simulink model "Drone_swarm_control"  (R2025a)
settings: Solver=FixedStepAuto  StartTime=0.0  StopTime=180  FixedStep=0.001  RelTol=1e-3
InitFcn:
  | %% Simulation parameters and waypoint trajectory
  | % Initial drone positions.
  | init_0=[0;0;0];
  | d_s=4;
  | init_1=init_0+d_s*[-1.1;0.1;0];
  | init_2=init_0+d_s*[0.3;-1.5;0];
  | init_3=init_0+d_s*[1.6;0.4;0];
  | init_4=init_0+d_s*[0.2;1.8;0];
  | 
  | % Initial battery energy in Wh.
  | E_0=77;
  | gain_2=1;
  | 
  | % PID controller gains.
  | PID_p=20;
  | PID_i=50;
  | PID_d=0;
  | 
  | % Router queues and background traffic.
  | router_buffer=160;
  | router_bandwith=300;
  | router_init_queue=[20,0,0,0,0];
  | traffic_mean=20;
  | traffic_variance=1;
  | 
  | % Communication-rate parameters.
  | F_max=2;
  | F_min=0.5;
  | F_H=(F_max+F_min)/3;
  | P_nc=(1-(F_H-F_min)/F_max);
  | 
  | 
  | % Desired formation offsets.
  | init_f_0=[0;0;0];
  | d_f=10;
  | init_f_1=init_0+d_f*[-1;0;0];
  | init_f_2=init_0+d_f*[0;-1;0];
  | init_f_3=init_0+d_f*[1;0;0];
  | init_f_4=init_0+d_f*[0;1;0];
  | 
  | 
  | % Waypoint mission with a fixed cruise altitude.
  | quota_fissa = -20;
  | 
  | waypoints = [
  |       0   0   0   0;
  |      75   0   quota_fissa   0;
  |     150   0   quota_fissa   0;
  |     225   0   quota_fissa   0;
  |     300   0   quota_fissa   0;
  |     300   0   quota_fissa   0;
  |     225  75   quota_fissa   0;
  |     150 150   quota_fissa   0;
  |      75 225   quota_fissa   0;
  |       0 300   quota_fissa   0;
  |       0 300   quota_fissa   0;
  |      75 300   quota_fissa   0;
  |     150 300   quota_fissa   0;
  |     225 300   quota_fissa   0;
  |     300 300   quota_fissa   0;
  |     300 300   quota_fissa   0;
  |     225 225   quota_fissa   0;
  |     150 150   quota_fissa   0;
  |      75  75   quota_fissa   0;
  |       0   0   quota_fissa   0;
  | ];
  | 
  | M = size(waypoints,1);
  | assert(M==20, &apos;You must supply exactly 20 waypoints.&apos;);
  | 
  | % Quadrotor mass and inertia.
  | mass = 1.2;
  | Ib   = diag([1.2416, 1.2416, 2*1.2416]);
  | 
  | % Mission duration and sampling interval.
  | ttot      = 3*60;
  | tdead     = 0;
  | totalTime = ttot + tdead;
  | % Time grid and waypoint trajectory.
  | Ts        = 0.001;
  | Nsamples  = round(totalTime/Ts) + 1;
  | t_sample  = linspace(0, totalTime, Nsamples);
  | 
  | % Waypoint dwell intervals used by the trajectory planner.
  | dwell    = 5;
  | Tflight  = ttot - M*dwell;
  | t_seg    = Tflight/(M-1);
  | 
  | % Repeat waypoint samples at arrival and departure times.
  | t_ext  = zeros(2*M,1);
  | wp_ext = zeros(2*M,4);
  | for i = 1:M
  |     t0             = (i-1)*(t_seg + dwell);
  |     t_ext(2*i-1)   = t0;
  |     t_ext(2*i)     = t0 + dwell;
  |     wp_ext(2*i-1,:)= waypoints(i,:);
  |     wp_ext(2*i,  :)= waypoints(i,:);
  | end
  | 
  | p_d      = zeros(4, Nsamples);
  | dot_p_d  = zeros(4, Nsamples);
  | ddot_p_d = zeros(4, Nsamples);
  | 
  | idx_traj = t_sample <= ttot;
  | t_active = t_sample(idx_traj);
  | 
  | % Build position and yaw splines with zero endpoint velocities.
  | for dim = 1:4
  |     pp   = spline(t_ext, [0, wp_ext(:,dim)&apos;, 0]);
  |     pp1  = fnder(pp,1);
  |     pp2  = fnder(pp,2);
  | 
  |     p_d(dim,    idx_traj) = ppval(pp,  t_active);
  |     dot_p_d(dim,idx_traj) = ppval(pp1, t_active);
  |     ddot_p_d(dim,idx_traj)= ppval(pp2, t_active);
  | end
  | 
  | % Hold the final waypoint during the optional settling interval.
  | if tdead>0
  |     last_wp = waypoints(end,:)&apos;;
  |     p_d(   :, ~idx_traj) = repmat(last_wp, 1, sum(~idx_traj));
  |     dot_p_d(:, ~idx_traj) = 0;
  |     ddot_p_d(:,~idx_traj) = 0;
  | end
  | 
  | % Reference signals used by the Simulink blocks.
  | csi_d      = p_d(1:3, :);
  | psi_d      = p_d(4,   :);
  | dot_csi_d  = dot_p_d(1:3, :);
  | ddot_csi_d = ddot_p_d(1:3, :);
  | dot_psi_d  = dot_p_d(4,   :);
  | ddot_psi_d = ddot_p_d(4,   :);
  | 
  | pos_0     = waypoints(1,1:3);
  | lin_vel_0 = [0 0 0];
  | w_bb_0    = [0 0 0];
  | 
  | 
  | t=t_sample;
undefined symbols (not defined in the file): A_diacenza, DiscIntNeverNeededParam, L
libraries: dspsigops x10, robotcorelib x5, slpidlib x5, dspstat3 x5, simulink x1, uavutilslib x1
(part 1 of 4)
settings Model: Creator=fabioruggiero  LastModifiedBy=tehen
settings ModelReferenceCC: EnableRefExpFcnMdlSchedulingChecks=on
settings RTWCC: GPUComputeCapability=3.5

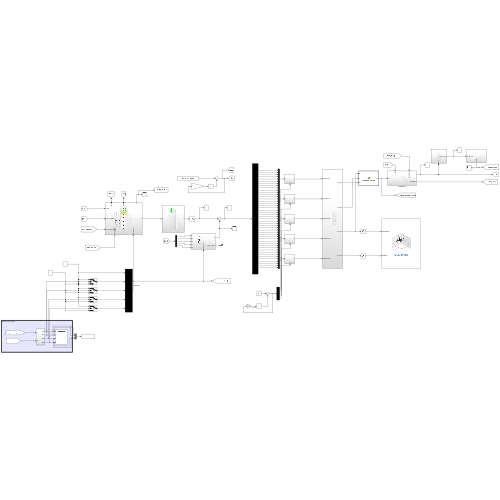
[thumbnail: Simulink's stored preview of the top-level diagram]
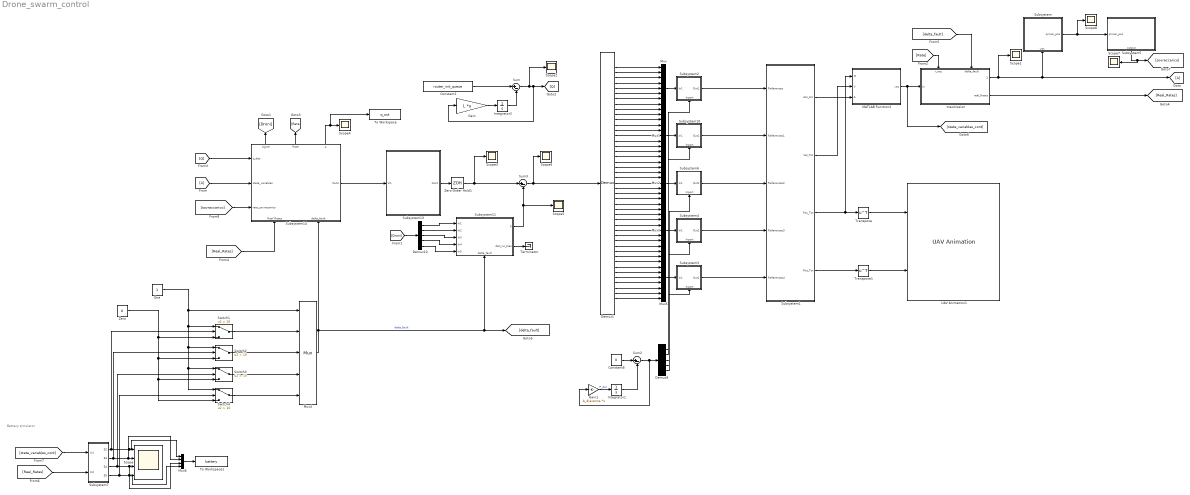
== system Drone_swarm_control ==
  note: Battery simulator
  Constant1 : Constant  Value=router_init_queue
  Constant8 : Constant  Value=0
  Demux1 : Demux  Outputs=45
  Demux10 : Demux  Outputs=5
  Demux9 : Demux  Outputs=5
  From : From
  Gain : Gain  Gain=L  Multiplication=Matrix(K*u)
  Gain1 : Gain  Gain=A_diacenza  Multiplication=Matrix(K*u)
  Goto : Goto
  Integrator1 : Integrator
  Integrator2 : Integrator
  MATLAB Function2 : MATLAB Function  TreatAsAtomicUnit=on
  Mux{,1..3,5} (5 alike) : Mux  Inputs=9
  Mux4 : Mux  Inputs=5
  Mux6 : Mux
  One : Constant  OutDataTypeStr=Inherit: Inherit via back propagation
  Scope : Scope  NumInputPorts=4
      settings: ActiveDisplayYMinimum=73.268572963914167  ActiveDisplayYMaximum=77.414603004009535  DataLoggingVariableName=ScopeData36
  Scope{1..8} (8 alike) : Scope
      Scope1 settings: ActiveDisplayYMinimum=-2.8153611493220492  ActiveDisplayYMaximum=3.6120762005014342  DataLoggingVariableName=ScopeData33
      Scope2 settings: ActiveDisplayYMinimum=-0.80480947223759247  ActiveDisplayYMaximum=7.2432852501383342  DataLoggingVariableName=ScopeData34
      Scope3 settings: ActiveDisplayYMinimum=-143.81794768951772  ActiveDisplayYMaximum=72.930943180534939  DataLoggingVariableName=ScopeData22
      Scope4 settings: ActiveDisplayYMinimum=-19.999999999999996  ActiveDisplayYMaximum=180  DataLoggingVariableName=ScopeData10
      Scope5 settings: ActiveDisplayYMinimum=-31.295142586026412  ActiveDisplayYMaximum=31.13864534366818  DataLoggingVariableName=ScopeData26
      Scope6 settings: ActiveDisplayYMinimum=-63.285546446382227  ActiveDisplayYMaximum=68.103390325053155  DataLoggingVariableName=ScopeData30
      Scope7 settings: ActiveDisplayYMinimum=-1  ActiveDisplayYMaximum=1  DataLoggingVariableName=ScopeData45
      Scope8 settings: ActiveDisplayYMinimum=-34.410281468941783  ActiveDisplayYMaximum=109.69253321204845  DataLoggingVariableName=ScopeData38
  Subsystem : Subsystem
      settings: PortSchema="{\"entries\":[{\"content\":{\"sides\":[{\"content\":{},\"type\":\"ConnectorPlacement.EquallySpacedRectSide\",\"uuid\":\"08878166-f0fb-4fb4-8499-3220f0500d52\"},{\"content\":{\"connectorIds\":[\"Out1\"],\"side\":\"RIGHT\"},\"type\":\"ConnectorPlacement.EquallySpacedRectSide\",\"uuid\":\"3c5bd1ef-4402-434f-96a9-2e68d96c1f89\"},{\"content\":{\"side\":\"TOP\"},\"type\":\"ConnectorPlacement.EquallySpacedRectSide\",\"uuid\":\"fffe2cbe-d1b2-4ad1-ad76-24284be8719f\"},{\"content\":{\"connectorIds\":[\"In1\"],\"side\":\"BOTTOM\"},\"type\":\"ConnectorPlacement.EquallySpacedRectSide\",\"uuid\":\"822b8eda-48e8-4a99-8864-f0043c7d4993\"}]},\"type\":\"ConnectorPlacement.EquallySpacedConnector\",\"uuid\":\"fdf8a493-4def-4212-9b4e-e4f95273dccb\"}],\"packageUris\":[\"http://schema.mathworks.com/mf0/Connector/R2020b\"],\"version\":\"1.0\"}"
  Subsystem1 : Subsystem
  Subsystem10 : Subsystem
      settings: PortSchema="{\"entries\":[{\"content\":{\"sides\":[{\"content\":{\"connectorIds\":[\"In1\"]},\"type\":\"ConnectorPlacement.EquallySpacedRectSide\",\"uuid\":\"6e5d8b99-8054-458f-abbe-7e3d6126420c\"},{\"content\":{\"connectorIds\":[\"Out1\"],\"side\":\"RIGHT\"},\"type\":\"ConnectorPlacement.EquallySpacedRectSide\",\"uuid\":\"d8af8c34-1227-4a19-bfdc-b42d943ed13c\"},{\"content\":{\"side\":\"TOP\"},\"type\":\"ConnectorPlacement.EquallySpacedRectSide\",\"uuid\":\"9c10b933-2873-4349-b535-f2af5c16ec70\"},{\"content\":{\"connectorIds\":[\"In2\"],\"side\":\"BOTTOM\"},\"type\":\"ConnectorPlacement.EquallySpacedRectSide\",\"uuid\":\"05be8d01-ed26-4f96-bcb1-0e501cb43bcc\"}]},\"type\":\"ConnectorPlacement.EquallySpacedConnector\",\"uuid\":\"f87e25de-488b-44c6-b2e5-9d22d609821c\"}],\"packageUris\":[\"http://schema.mathworks.com/mf0/Connector/R2020b\"],\"version\":\"1.0\"}"
  Subsystem11 : Subsystem
      settings: PortSchema="{\"entries\":[{\"content\":{\"sides\":[{\"content\":{\"connectorIds\":[\"In1\",\"In2\",\"In3\",\"In4\",\"In5\"]},\"type\":\"ConnectorPlacement.EquallySpacedRectSide\",\"uuid\":\"82243081-7292-4dd7-bbb8-2b3f3ffda34e\"},{\"content\":{\"connectorIds\":[\"Out1\",\"Out2\"],\"side\":\"RIGHT\"},\"type\":\"ConnectorPlacement.EquallySpacedRectSide\",\"uuid\":\"0c768998-383c-4b1c-86c0-02766a2c634a\"},{\"content\":{\"side\":\"TOP\"},\"type\":\"ConnectorPlacement.EquallySpacedRectSide\",\"uuid\":\"2d16c04a-7161-4b14-a0bc-a057e1fb9d07\"},{\"content\":{\"connectorIds\":[\"In6\"],\"side\":\"BOTTOM\"},\"type\":\"ConnectorPlacement.EquallySpacedRectSide\",\"uuid\":\"700b63a7-d9a8-4585-a364-11c2f92fed84\"}]},\"type\":\"ConnectorPlacement.EquallySpacedConnector\",\"uuid\":\"2c45eea6-509d-46c9-bd27-2690d9a9f219\"}],\"packageUris\":[\"http://schema.mathworks.com/mf0/Connector/R2020b\"],\"version\":\"1.0\"}"
  Subsystem13 : Subsystem
  Subsystem14 : Subsystem
      settings: PortSchema="{\"entries\":[{\"content\":{\"sides\":[{\"content\":{\"connectorIds\":[\"In1\",\"In2\",\"In3\"]},\"type\":\"ConnectorPlacement.EquallySpacedRectSide\",\"uuid\":\"f1d046dc-675d-4db9-bf29-bca78bce001f\"},{\"content\":{\"connectorIds\":[\"Out1\"],\"side\":\"RIGHT\"},\"type\":\"ConnectorPlacement.EquallySpacedRectSide\",\"uuid\":\"811f6c37-e862-4f2b-bd7d-8070e0d60dff\"},{\"content\":{\"connectorIds\":[\"Out2\",\"Out3\",\"Out4\"],\"side\":\"TOP\"},\"type\":\"ConnectorPlacement.EquallySpacedRectSide\",\"uuid\":\"cf9e60f1-1ac0-454e-9388-0113fe782dd3\"},{\"content\":{\"connectorIds\":[\"In4\",\"In5\"],\"side\":\"BOTTOM\"},\"type\":\"ConnectorPlacement.EquallySpacedRectSide\",\"uuid\":\"1705a36f-5e80-44a6-ab31-ad29025d66f8\"}]},\"type\":\"ConnectorPlacement.EquallySpacedConnector\",\"uuid\":\"a6589967-962b-441c-ab9d-1a23d8667ece\"}],\"packageUris\":[\"http://schema.mathworks.com/mf0/Connector/R2020b\"],\"version\":\"1.0\"}"
  Subsystem2 : Subsystem
      settings: PortSchema="{\"entries\":[{\"content\":{\"sides\":[{\"content\":{\"connectorIds\":[\"In1\"]},\"type\":\"ConnectorPlacement.EquallySpacedRectSide\",\"uuid\":\"6e5d8b99-8054-458f-abbe-7e3d6126420c\"},{\"content\":{\"connectorIds\":[\"Out1\"],\"side\":\"RIGHT\"},\"type\":\"ConnectorPlacement.EquallySpacedRectSide\",\"uuid\":\"d8af8c34-1227-4a19-bfdc-b42d943ed13c\"},{\"content\":{\"side\":\"TOP\"},\"type\":\"ConnectorPlacement.EquallySpacedRectSide\",\"uuid\":\"9c10b933-2873-4349-b535-f2af5c16ec70\"},{\"content\":{\"connectorIds\":[\"In2\"],\"side\":\"BOTTOM\"},\"type\":\"ConnectorPlacement.EquallySpacedRectSide\",\"uuid\":\"05be8d01-ed26-4f96-bcb1-0e501cb43bcc\"}]},\"type\":\"ConnectorPlacement.EquallySpacedConnector\",\"uuid\":\"f87e25de-488b-44c6-b2e5-9d22d609821c\"}],\"packageUris\":[\"http://schema.mathworks.com/mf0/Connector/R2020b\"],\"version\":\"1.0\"}"
  Subsystem3 : Subsystem
      settings: PortSchema="{\"entries\":[{\"content\":{\"sides\":[{\"content\":{\"connectorIds\":[\"In1\"]},\"type\":\"ConnectorPlacement.EquallySpacedRectSide\",\"uuid\":\"6e5d8b99-8054-458f-abbe-7e3d6126420c\"},{\"content\":{\"connectorIds\":[\"Out1\"],\"side\":\"RIGHT\"},\"type\":\"ConnectorPlacement.EquallySpacedRectSide\",\"uuid\":\"d8af8c34-1227-4a19-bfdc-b42d943ed13c\"},{\"content\":{\"side\":\"TOP\"},\"type\":\"ConnectorPlacement.EquallySpacedRectSide\",\"uuid\":\"9c10b933-2873-4349-b535-f2af5c16ec70\"},{\"content\":{\"connectorIds\":[\"In2\"],\"side\":\"BOTTOM\"},\"type\":\"ConnectorPlacement.EquallySpacedRectSide\",\"uuid\":\"05be8d01-ed26-4f96-bcb1-0e501cb43bcc\"}]},\"type\":\"ConnectorPlacement.EquallySpacedConnector\",\"uuid\":\"f87e25de-488b-44c6-b2e5-9d22d609821c\"}],\"packageUris\":[\"http://schema.mathworks.com/mf0/Connector/R2020b\"],\"version\":\"1.0\"}"
  Subsystem4 : Subsystem
      settings: PortSchema="{\"entries\":[{\"content\":{\"sides\":[{\"content\":{\"connectorIds\":[\"In1\"]},\"type\":\"ConnectorPlacement.EquallySpacedRectSide\",\"uuid\":\"6e5d8b99-8054-458f-abbe-7e3d6126420c\"},{\"content\":{\"connectorIds\":[\"Out1\"],\"side\":\"RIGHT\"},\"type\":\"ConnectorPlacement.EquallySpacedRectSide\",\"uuid\":\"d8af8c34-1227-4a19-bfdc-b42d943ed13c\"},{\"content\":{\"side\":\"TOP\"},\"type\":\"ConnectorPlacement.EquallySpacedRectSide\",\"uuid\":\"9c10b933-2873-4349-b535-f2af5c16ec70\"},{\"content\":{\"connectorIds\":[\"In2\"],\"side\":\"BOTTOM\"},\"type\":\"ConnectorPlacement.EquallySpacedRectSide\",\"uuid\":\"05be8d01-ed26-4f96-bcb1-0e501cb43bcc\"}]},\"type\":\"ConnectorPlacement.EquallySpacedConnector\",\"uuid\":\"f87e25de-488b-44c6-b2e5-9d22d609821c\"}],\"packageUris\":[\"http://schema.mathworks.com/mf0/Connector/R2020b\"],\"version\":\"1.0\"}"
  Subsystem5 : Subsystem
      settings: PortSchema="{\"entries\":[{\"content\":{\"sides\":[{\"content\":{},\"type\":\"ConnectorPlacement.EquallySpacedRectSide\",\"uuid\":\"08878166-f0fb-4fb4-8499-3220f0500d52\"},{\"content\":{\"connectorIds\":[\"Out1\"],\"side\":\"RIGHT\"},\"type\":\"ConnectorPlacement.EquallySpacedRectSide\",\"uuid\":\"3c5bd1ef-4402-434f-96a9-2e68d96c1f89\"},{\"content\":{\"side\":\"TOP\"},\"type\":\"ConnectorPlacement.EquallySpacedRectSide\",\"uuid\":\"fffe2cbe-d1b2-4ad1-ad76-24284be8719f\"},{\"content\":{\"connectorIds\":[\"In1\"],\"side\":\"BOTTOM\"},\"type\":\"ConnectorPlacement.EquallySpacedRectSide\",\"uuid\":\"822b8eda-48e8-4a99-8864-f0043c7d4993\"}]},\"type\":\"ConnectorPlacement.EquallySpacedConnector\",\"uuid\":\"fdf8a493-4def-4212-9b4e-e4f95273dccb\"}],\"packageUris\":[\"http://schema.mathworks.com/mf0/Connector/R2020b\"],\"version\":\"1.0\"}"
  Subsystem6 : Subsystem
      settings: PortSchema="{\"entries\":[{\"content\":{\"sides\":[{\"content\":{\"connectorIds\":[\"In1\"]},\"type\":\"ConnectorPlacement.EquallySpacedRectSide\",\"uuid\":\"6e5d8b99-8054-458f-abbe-7e3d6126420c\"},{\"content\":{\"connectorIds\":[\"Out1\"],\"side\":\"RIGHT\"},\"type\":\"ConnectorPlacement.EquallySpacedRectSide\",\"uuid\":\"d8af8c34-1227-4a19-bfdc-b42d943ed13c\"},{\"content\":{\"side\":\"TOP\"},\"type\":\"ConnectorPlacement.EquallySpacedRectSide\",\"uuid\":\"9c10b933-2873-4349-b535-f2af5c16ec70\"},{\"content\":{\"connectorIds\":[\"In2\"],\"side\":\"BOTTOM\"},\"type\":\"ConnectorPlacement.EquallySpacedRectSide\",\"uuid\":\"05be8d01-ed26-4f96-bcb1-0e501cb43bcc\"}]},\"type\":\"ConnectorPlacement.EquallySpacedConnector\",\"uuid\":\"f87e25de-488b-44c6-b2e5-9d22d609821c\"}],\"packageUris\":[\"http://schema.mathworks.com/mf0/Connector/R2020b\"],\"version\":\"1.0\"}"
  Subsystem7 : Subsystem
  Sum : Sum  Inputs=|+-
  Sum2 : Sum  Inputs=|+-
  Sum3 : Sum  Inputs=|+-
  Switch{1..4} (4 alike) : Switch  Criteria=u2 > Threshold  Threshold=10  SaturateOnIntegerOverflow=off  InputSameDT=off
  Terminator : Terminator
  To Workspace : ToWorkspace  VariableName=q_out  SaveFormat=Timeseries  SampleTime=-1
  To Workspace1 : ToWorkspace  VariableName=battery  SaveFormat=Timeseries  SampleTime=-1
  Transpose : Math  Operator=transpose
  Transpose1 : Math  Operator=transpose
  UAV Animation1 : uavutilslib/UAV Animation  NumUAV=5  DynamicUAVConfig=off  UAVType=Multirotor  UAVSize=1  UAVColor=[1 0 0]  UAVTrajectoryAlpha=1  InertialZDirection=Down  RotationFormat=Quaternion  DrawMarkers=off  SampleTime=0.1
  Zero : Constant  Value=0  OutDataTypeStr=Inherit: Inherit via back propagation
  Zero-Order Hold1 : ZeroOrderHold  SampleTime=-1
  trasmission : Subsystem
      settings: PortSchema="{\"entries\":[{\"content\":{\"sides\":[{\"content\":{\"connectorIds\":[\"In1\"]},\"type\":\"ConnectorPlacement.EquallySpacedRectSide\",\"uuid\":\"4dfdb4a7-0a88-4bc0-a7e6-6eaded6ab7ea\"},{\"content\":{\"connectorIds\":[\"Out1\",\"Out2\"],\"side\":\"RIGHT\"},\"type\":\"ConnectorPlacement.EquallySpacedRectSide\",\"uuid\":\"9b9e2090-1e21-4d2a-8a8a-73b93d842d99\"},{\"content\":{\"connectorIds\":[\"In2\",\"In3\"],\"side\":\"TOP\"},\"type\":\"ConnectorPlacement.EquallySpacedRectSide\",\"uuid\":\"40eb9426-960b-4b19-8bb6-92ef73d2d0da\"}]},\"type\":\"ConnectorPlacement.EquallySpacedConnector\",\"uuid\":\"8e0959b2-0aca-4b3e-87b3-3e8255b5da73\"}],\"packageUris\":[\"http://schema.mathworks.com/mf0/Connector/R2020b\"],\"version\":\"1.0\"}"
  wires:
  Demux9/5 -> Subsystem3/2(Inport)
  Transpose1/1 -> UAV Animation1/2
  Transpose/1 -> UAV Animation1/1
  Sum2/1 -> Demux9/1, Gain1/1
  Gain1/1 -> Integrator1/1  "P_dot"
  Integrator1/1 -> Sum2/2
  Mux3/1 -> Subsystem4/1(In1)
  Mux/1 -> Subsystem2/1(In1)
  Subsystem2/1(Out1) -> Subsystem1/1(References)
  Demux9/2 -> Subsystem10/2(Inport)
  Subsystem3/1(Out1) -> Subsystem1/5(References4)
  Mux5/1 -> Subsystem3/1(In1)
  Subsystem6/1(Out1) -> Subsystem1/3(References2)
  Mux2/1 -> Subsystem6/1(In1)
  Demux1/1 -> Mux/1
  Demux1/15 -> Mux1/6
  Demux9/1 -> Subsystem2/2(Inport)
  Demux1/23 -> Mux2/5
  Demux1/12 -> Mux1/3
  Demux1/4 -> Mux/4
  Demux1/31 -> Mux3/4
  Demux1/41 -> Mux5/5
  Demux1/19 -> Mux2/1
  Demux1/26 -> Mux2/8
  Demux1/29 -> Mux3/2
  Demux1/34 -> Mux3/7
  Demux1/39 -> Mux5/3
  Demux1/20 -> Mux2/2
  Demux1/38 -> Mux5/2
  Demux1/43 -> Mux5/7
  Demux1/42 -> Mux5/6
  Demux1/30 -> Mux3/3
  Demux1/36 -> Mux3/9
  Demux1/27 -> Mux2/9
  Demux9/4 -> Subsystem4/2(Inport)
  Demux1/22 -> Mux2/4
  Demux1/32 -> Mux3/5
  Demux1/14 -> Mux1/5
  Demux1/13 -> Mux1/4
  Demux1/21 -> Mux2/3
  Demux1/33 -> Mux3/6
  Subsystem1/4(Rot_Tot) -> Transpose1/1
  Demux1/9 -> Mux/9
  Mux1/1 -> Subsystem10/1(In1)
  Demux1/40 -> Mux5/4
  Demux1/3 -> Mux/3
  Demux1/6 -> Mux/6
  Demux1/25 -> Mux2/7
  Demux1/8 -> Mux/8
  Demux1/28 -> Mux3/1
  Demux1/10 -> Mux1/1
  Demux1/7 -> Mux/7
  Demux1/37 -> Mux5/1
  Demux1/11 -> Mux1/2
  Demux1/45 -> Mux5/9
  Demux1/17 -> Mux1/8
  Demux1/35 -> Mux3/8
  Demux1/5 -> Mux/5
  Demux1/44 -> Mux5/8
  Demux1/18 -> Mux1/9
  Demux1/16 -> Mux1/7
  Demux1/2 -> Mux/2
  Constant8/1 -> Sum2/1
  Subsystem4/1(Out1) -> Subsystem1/4(References3)
  Demux9/3 -> Subsystem6/2(Inport)
  Demux1/24 -> Mux2/6
  Subsystem10/1(Out1) -> Subsystem1/2(References1)
  Subsystem1/3(Pos_Tot) -> Transpose/1, MATLAB Function2/1(M)
  Subsystem1/2(Vel_Tot) -> MATLAB Function2/2(V)
  Subsystem1/1(Acc_tot) -> MATLAB Function2/3(A)
  Subsystem11/1(P) -> Scope5/1, Sum3/2
  Demux10/1 -> Subsystem11/1(In1)
  Demux10/2 -> Subsystem11/2(In2)
  Demux10/3 -> Subsystem11/3(In3)
  Demux10/4 -> Subsystem11/4(In4)
  Demux10/5 -> Subsystem11/5(In5)
  [Droni] -> Demux10/1
  Gain/1 -> Integrator2/1
  Constant1/1 -> Sum/1
  MATLAB Function2/1(vec) -> [state_variables_cont], trasmission/1(In)
  [Rate] -> trasmission/2(r_req)
  [Q] -> Subsystem14/1(q_des)
  From/1 -> Subsystem14/2(state_variables)
  Subsystem14/2(signal) -> [Droni]
  Subsystem14/3(Rate) -> [Rate]
  Subsystem14/1(Out4) -> Subsystem13/1(In1)
  trasmission/2(real_Rates) -> [Real_Rates]
  [Real_Rates] -> Subsystem14/4(" Real Rates")
  Integrator2/1 -> Sum/2
  Sum/1 -> Scope2/1, [Q], Gain/1
  Subsystem14/4(q) -> To Workspace/1, Scope4/1
  Subsystem13/1(Out1) -> Zero-Order Hold1/1
  Zero-Order Hold1/1 -> Scope3/1, Sum3/1
  Mux4/1 -> Subsystem14/5(delta_fault), [delta_fault], Subsystem11/6(delta_fault)  "delta_fault"
  [delta_fault] -> trasmission/3(delta_fault)
  Sum3/1 -> Demux1/1, Scope6/1
  [state_variables_cont] -> Subsystem7/1(In1)
  [Real_Rates] -> Subsystem7/2(In2)
  Subsystem7/1(E2) -> Switch1/2, Mux6/1, Scope/1
  Subsystem7/2(E3) -> Switch2/2, Mux6/2, Scope/2
  Subsystem7/3(E4) -> Mux6/3, Scope/3, Switch3/2
  Subsystem7/4(E5) -> Mux6/4, Scope/4, Switch4/2
  Subsystem11/2(dati_no_bias) -> Terminator/1
  trasmission/1(" ") -> Goto/1, Subsystem/1(vec), Scope1/1
  Subsystem/1(pinner_pos) -> Scope8/1, Subsystem5/1(pinner_pos)
  Subsystem5/1(output) -> Scope7/1, [sovraccarico]
  [sovraccarico] -> Subsystem14/3("rate_sovraccarico ")
  Mux6/1 -> To Workspace1/1
  Switch1/1 -> Mux4/2
  Switch2/1 -> Mux4/3
  Switch3/1 -> Mux4/4
  Switch4/1 -> Mux4/5
  One/1 -> Mux4/1, Switch4/1, Switch3/1, Switch2/1, Switch1/1
  Zero/1 -> Switch4/3, Switch3/3, Switch2/3, Switch1/3

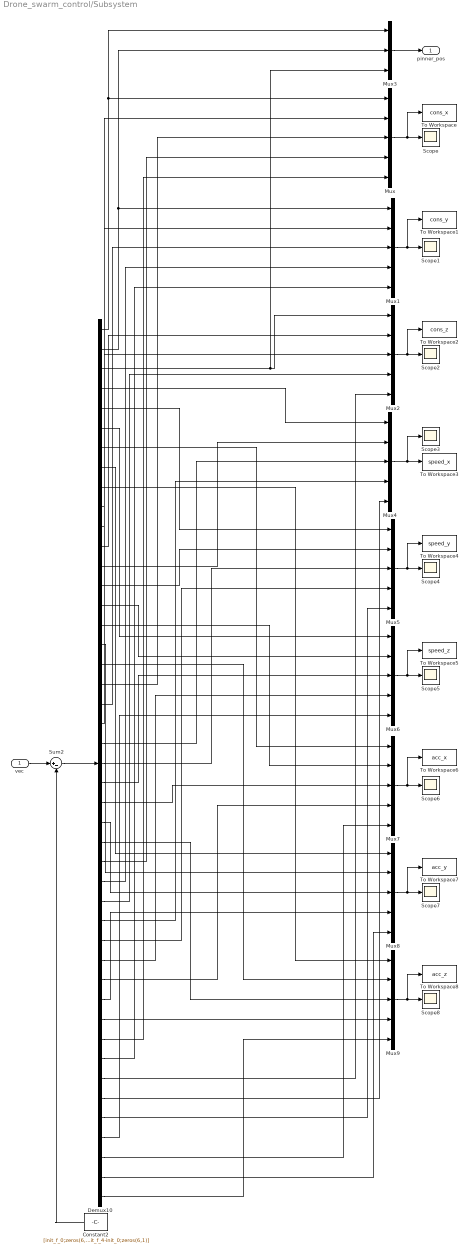
== system Drone_swarm_control/Subsystem ==
  vec : Inport
  Constant2 : Constant  Value=[init_f_0;zeros(6,1);init_f_1-init_0;zeros(6,1);init_f_2-init_0;zeros(6,1);init_f_3-init_0;zeros(6,1);init_f_4-init_0;zeros(6,1)]
  Demux10 : Demux  Outputs=45
  Mux{,1..2,4..9} (9 alike) : Mux  Inputs=5
  Mux3 : Mux  Inputs=3
  Scope{,1..8} (9 alike) : Scope
      Scope settings: ActiveDisplayYMinimum=-5.0339863966909171  ActiveDisplayYMaximum=4.70331510038157  DataLoggingVariableName=ScopeData8
      Scope1 settings: ActiveDisplayYMinimum=-7.6500004579712169  ActiveDisplayYMaximum=8.8500005655108129  DataLoggingVariableName=ScopeData9
      Scope2 settings: ActiveDisplayYMinimum=-20.5736  ActiveDisplayYMaximum=0.39733  DataLoggingVariableName=ScopeData10
      Scope3 settings: ActiveDisplayYMinimum=-12.5  ActiveDisplayYMaximum=12.5  DataLoggingVariableName=ScopeData35
      Scope4 settings: ActiveDisplayYMinimum=-10.922558607915478  ActiveDisplayYMaximum=12.324728734212831  DataLoggingVariableName=ScopeData39
      Scope5 settings: ActiveDisplayYMinimum=-20.5736  ActiveDisplayYMaximum=0.39733  DataLoggingVariableName=ScopeData40
      Scope6 settings: ActiveDisplayYMinimum=-5.0339863966909171  ActiveDisplayYMaximum=4.70331510038157  DataLoggingVariableName=ScopeData41
      Scope7 settings: ActiveDisplayYMinimum=-5.0339863966909171  ActiveDisplayYMaximum=4.70331510038157  DataLoggingVariableName=ScopeData42
      Scope8 settings: ActiveDisplayYMinimum=-5.0339863966909171  ActiveDisplayYMaximum=4.70331510038157  DataLoggingVariableName=ScopeData43
  Sum2 : Sum  Inputs=|+-
  To Workspace : ToWorkspace  VariableName=cons_x  SaveFormat=Structure With Time  SampleTime=-1
  To Workspace1 : ToWorkspace  VariableName=cons_y  SaveFormat=Structure With Time  SampleTime=-1
  To Workspace2 : ToWorkspace  VariableName=cons_z  SaveFormat=Structure With Time  SampleTime=-1
  To Workspace3 : ToWorkspace  VariableName=speed_x  SaveFormat=Structure With Time  SampleTime=-1
  To Workspace4 : ToWorkspace  VariableName=speed_y  SaveFormat=Structure With Time  SampleTime=-1
  To Workspace5 : ToWorkspace  VariableName=speed_z  SaveFormat=Structure With Time  SampleTime=-1
  To Workspace6 : ToWorkspace  VariableName=acc_x  SaveFormat=Structure With Time  SampleTime=-1
  To Workspace7 : ToWorkspace  VariableName=acc_y  SaveFormat=Structure With Time  SampleTime=-1
  To Workspace8 : ToWorkspace  VariableName=acc_z  SaveFormat=Structure With Time  SampleTime=-1
  pinner_pos : Outport
  wires:
  Demux10/13 -> Mux4/2
  Demux10/5 -> Mux5/1
  Demux10/20 -> Mux1/3
  Demux10/12 -> Mux2/2
  vec/1 -> Sum2/1
  Demux10/4 -> Mux4/1
  Demux10/19 -> Mux/3
  Demux10/11 -> Mux1/2
  Demux10/3 -> Mux3/3, Mux2/1
  Demux10/18 -> Mux9/2
  Demux10/10 -> Mux/2
  Demux10/2 -> Mux1/1, Mux3/2
  Demux10/17 -> Mux8/2
  Demux10/9 -> Mux9/1
  Demux10/1 -> Mux3/1, Mux/1
  Demux10/14 -> Mux5/2
  Demux10/6 -> Mux6/1
  Constant2/1 -> Sum2/2
  Mux2/1 -> Scope2/1, To Workspace2/1
  Sum2/1 -> Demux10/1
  Demux10/15 -> Mux6/2
  Demux10/7 -> Mux7/1
  Demux10/16 -> Mux7/2
  Demux10/8 -> Mux8/1
  Demux10/45 -> Mux9/5
  Demux10/37 -> Mux/5
  Demux10/29 -> Mux1/4
  Demux10/21 -> Mux2/3
  Demux10/38 -> Mux1/5
  Demux10/30 -> Mux2/4
  Demux10/22 -> Mux4/3
  Demux10/39 -> Mux2/5
  Demux10/31 -> Mux4/4
  Demux10/23 -> Mux5/3
  Demux10/40 -> Mux4/5
  Demux10/32 -> Mux5/4
  Demux10/24 -> Mux6/3
  Demux10/41 -> Mux5/5
  Demux10/33 -> Mux6/4
  Demux10/25 -> Mux7/3
  Demux10/42 -> Mux6/5
  Demux10/34 -> Mux7/4
  Demux10/26 -> Mux8/3
  Mux/1 -> Scope/1, To Workspace/1
  Demux10/43 -> Mux7/5
  Demux10/35 -> Mux8/4
  Demux10/27 -> Mux9/3
  Demux10/44 -> Mux8/5
  Demux10/36 -> Mux9/4
  Demux10/28 -> Mux/4
  Mux3/1 -> pinner_pos/1
  Mux1/1 -> Scope1/1, To Workspace1/1
  Mux4/1 -> Scope3/1, To Workspace3/1
  Mux5/1 -> Scope4/1, To Workspace4/1
  Mux6/1 -> To Workspace5/1, Scope5/1
  Mux7/1 -> To Workspace6/1, Scope6/1
  Mux8/1 -> Scope7/1, To Workspace7/1
  Mux9/1 -> To Workspace8/1, Scope8/1

== system Drone_swarm_control/Subsystem1 ==
  References : Inport
  References1 : Inport  Port=2
  References2 : Inport  Port=3
  References3 : Inport  Port=4
  References4 : Inport  Port=5
  Saturation : Saturate  UpperLimit=10  LowerLimit=-10
  Subsystem : Subsystem
  Subsystem1 : Subsystem
  Subsystem2 : Subsystem
  Subsystem3 : Subsystem
  Subsystem_1 : Subsystem
  Subsystem_2 : Subsystem
  Subsystem_3 : Subsystem
  Subsystem_4 : Subsystem
  Subsystem_5 : Subsystem
  Acc_tot : Outport
  Vel_Tot : Outport  Port=2
  Pos_Tot : Outport  Port=3
  Rot_Tot : Outport  Port=4
  wires:
  References1/1 -> Subsystem_2/1(References)
  References2/1 -> Subsystem_3/1(References)
  References3/1 -> Subsystem_4/1(References)
  References/1 -> Subsystem_1/1(References)
  References4/1 -> Subsystem_5/1(References)
  Subsystem_1/2(Lin Vel) -> Subsystem/1(In1)
  Subsystem_2/2(Lin Vel) -> Subsystem/2(In2)
  Subsystem_3/2(Lin Vel) -> Subsystem/3(In3)
  Subsystem_4/2(Lin Vel) -> Subsystem/4(In4)
  Subsystem_5/2(Lin Vel) -> Subsystem/5(In5)
  Subsystem/1(Out1) -> Saturation/1
  Subsystem_1/3(Lin Pos) -> Subsystem1/1(In1)
  Subsystem_2/3(Lin Pos) -> Subsystem1/2(In2)
  Subsystem_3/3(Lin Pos) -> Subsystem1/3(In3)
  Subsystem_4/3(Lin Pos) -> Subsystem1/4(In4)
  Subsystem_5/3(Lin Pos) -> Subsystem1/5(In5)
  Subsystem1/1(Out1) -> Pos_Tot/1
  Subsystem_1/4(Rotation) -> Subsystem2/1(In1)
  Subsystem_2/4(Rotation) -> Subsystem2/2(In2)
  Subsystem_3/4(Rotation) -> Subsystem2/3(In3)
  Subsystem_4/4(Rotation) -> Subsystem2/4(In4)
  Subsystem_5/4(Rotation) -> Subsystem2/5(In5)
  Subsystem2/1(Out1) -> Rot_Tot/1
  Subsystem_1/1(Lin Acc) -> Subsystem3/1(In1)
  Subsystem_2/1(Lin Acc) -> Subsystem3/2(In2)
  Subsystem_3/1(Lin Acc) -> Subsystem3/3(In3)
  Subsystem_4/1(Lin Acc) -> Subsystem3/4(In4)
  Subsystem_5/1(Lin Acc) -> Subsystem3/5(In5)
  Subsystem3/1(Out1) -> Acc_tot/1
  Saturation/1 -> Vel_Tot/1

== system Drone_swarm_control/Subsystem10 ==
  In1 : Inport
  Inport : Inport  Port=2
  Constant1 : Constant  Value=[0;0;0]
  Demux : Demux  Outputs=9
  Demux1 : Demux  Outputs=3
  Mux : Mux  Inputs=3
  Mux2 : Mux  Inputs=10
  Sum : Sum  Inputs=++|
  Out1 : Outport
  wires:
  Mux2/1 -> Out1/1
  In1/1 -> Demux/1
  Demux/4 -> Mux2/4
  Demux/5 -> Mux2/5
  Demux/6 -> Mux2/6
  Demux/7 -> Mux2/7
  Demux/8 -> Mux2/8
  Demux/9 -> Mux2/9
  Demux/1 -> Mux/1
  Demux/2 -> Mux/2
  Demux/3 -> Mux/3
  Mux/1 -> Sum/2
  Constant1/1 -> Sum/1
  Sum/1 -> Demux1/1
  Demux1/1 -> Mux2/1
  Demux1/2 -> Mux2/2
  Demux1/3 -> Mux2/3
  Inport/1 -> Mux2/10

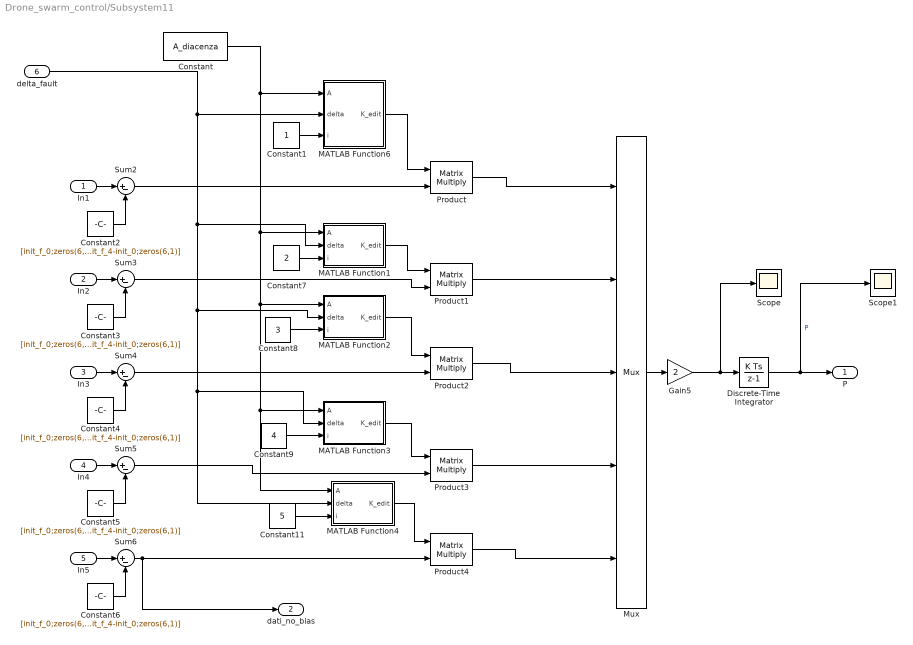
== system Drone_swarm_control/Subsystem11 ==
  In1 : Inport
  In2 : Inport  Port=2
  In3 : Inport  Port=3
  In4 : Inport  Port=4
  In5 : Inport  Port=5
  delta_fault : Inport  Port=6
  Constant : Constant  Value=A_diacenza
  Constant1 : Constant
  Constant11 : Constant  Value=5
  Constant{2..6} (5 alike) : Constant  Value=[init_f_0;zeros(6,1);init_f_1-init_0;zeros(6,1);init_f_2-init_0;zeros(6,1);init_f_3-init_0;zeros(6,1);init_f_4-init_0;zeros(6,1)]
  Constant7 : Constant  Value=2
  Constant8 : Constant  Value=3
  Constant9 : Constant  Value=4
  Discrete-Time Integrator : DiscreteIntegrator  SampleTime=-1  ICPrevOutput=DiscIntNeverNeededParam  ICPrevScaledInput=DiscIntNeverNeededParam
  Gain5 : Gain  Gain=2
  MATLAB Function1 : MATLAB Function  TreatAsAtomicUnit=on
  MATLAB Function2 : MATLAB Function  TreatAsAtomicUnit=on
  MATLAB Function3 : MATLAB Function  TreatAsAtomicUnit=on
  MATLAB Function4 : MATLAB Function  TreatAsAtomicUnit=on
  MATLAB Function6 : MATLAB Function  TreatAsAtomicUnit=on
  Mux : Mux  Inputs=5
  Product{,1..4} (5 alike) : Product  Multiplication=Matrix(*)
  Scope : Scope
      settings: ActiveDisplayYMinimum=-1  ActiveDisplayYMaximum=1  DataLoggingVariableName=ScopeData27
  Scope1 : Scope
      settings: ActiveDisplayYMinimum=-27.096024824890314  ActiveDisplayYMaximum=25.2419506186057  DataLoggingVariableName=ScopeData28
  Sum{2..6} (5 alike) : Sum  Inputs=|+-
  P : Outport
  dati_no_bias : Outport  Port=2
  wires:
  Discrete-Time Integrator/1 -> Scope1/1, P/1  "P"
  Constant2/1 -> Sum2/2
  Constant3/1 -> Sum3/2
  Constant4/1 -> Sum4/2
  Constant5/1 -> Sum5/2
  Constant6/1 -> Sum6/2
  Sum2/1 -> Product/2
  Mux/1 -> Gain5/1
  In1/1 -> Sum2/1
  In2/1 -> Sum3/1
  In3/1 -> Sum4/1
  In4/1 -> Sum5/1
  In5/1 -> Sum6/1
  Sum3/1 -> Product1/2
  Sum4/1 -> Product2/2
  Sum5/1 -> Product3/2
  Product1/1 -> Mux/2
  Product2/1 -> Mux/3
  Product3/1 -> Mux/4
  Product4/1 -> Mux/5
  Gain5/1 -> Discrete-Time Integrator/1, Scope/1
  delta_fault/1 -> MATLAB Function4/2(delta), MATLAB Function3/2(delta), MATLAB Function2/2(delta), MATLAB Function1/2(delta), MATLAB Function6/2(delta)
  Constant1/1 -> MATLAB Function6/3(i)
  MATLAB Function6/1(K_edit) -> Product/1
  MATLAB Function4/1(K_edit) -> Product4/1
  MATLAB Function3/1(K_edit) -> Product3/1
  MATLAB Function2/1(K_edit) -> Product2/1
  MATLAB Function1/1(K_edit) -> Product1/1
  Constant7/1 -> MATLAB Function1/3(i)
  Constant8/1 -> MATLAB Function2/3(i)
  Constant9/1 -> MATLAB Function3/3(i)
  Constant11/1 -> MATLAB Function4/3(i)
  Constant/1 -> MATLAB Function2/1(A), MATLAB Function4/1(A), MATLAB Function3/1(A), MATLAB Function1/1(A), MATLAB Function6/1(A)
  Sum6/1 -> dati_no_bias/1, Product4/2
  Product/1 -> Mux/1

== system Drone_swarm_control/Subsystem13 ==
  In1 : Inport
  Constant{5,10..12} (4 alike) : Constant  Value=0
  Constant3 : Constant  Value=init_1
  Constant4 : Constant  Value=init_3
  Constant6 : Constant  Value=init_4
  Constant9 : Constant  Value=init_2
  Demux : Demux  Outputs=15
  Demux{2..8} (7 alike) : Demux  Outputs=3
  Mux4 : Mux  Inputs=45
  Planner : Subsystem
  Terminator{,1..3} (4 alike) : Terminator
  Out1 : Outport
  wires:
  Demux/10 -> Mux4/34
  Demux6/1 -> Mux4/4
  Mux4/1 -> Out1/1
  Demux6/2 -> Mux4/5
  Demux4/1 -> Mux4/28
  Constant10/1 -> Mux4/13, Mux4/15, Mux4/14
  Demux/15 -> Mux4/45
  Demux3/2 -> Mux4/20
  Demux5/3 -> Mux4/39
  Planner/3(linear_acceleration_des) -> Demux8/1
  Constant9/1 -> Demux3/1
  Demux/3 -> Terminator2/1
  Constant11/1 -> Mux4/31, Mux4/33, Mux4/32
  Demux8/3 -> Mux4/9
  Constant6/1 -> Demux5/1
  Constant12/1 -> Mux4/40, Mux4/41, Mux4/42
  Demux3/1 -> Mux4/19
  Demux6/3 -> Mux4/6
  Demux/6 -> Mux4/18
  Demux8/2 -> Mux4/8
  Demux/1 -> Terminator/1
  Demux5/1 -> Mux4/37
  Demux5/2 -> Mux4/38
  Demux2/3 -> Mux4/3
  In1/1 -> Demux/1
  Demux3/3 -> Mux4/21
  Demux/12 -> Mux4/36
  Demux4/3 -> Mux4/30
  Demux7/2 -> Mux4/11
  Constant5/1 -> Mux4/22, Mux4/24, Mux4/23
  Demux/13 -> Mux4/43
  Constant3/1 -> Demux7/1
  Demux2/2 -> Mux4/2
  Demux/9 -> Mux4/27
  Demux7/3 -> Mux4/12
  Demux/4 -> Mux4/16
  Demux/8 -> Mux4/26
  Planner/4(xb_des) -> Terminator3/1
  Demux/14 -> Mux4/44
  Demux2/1 -> Mux4/1
  Demux/7 -> Mux4/25
  Demux/2 -> Terminator1/1
  Demux/5 -> Mux4/17
  Demux8/1 -> Mux4/7
  Constant4/1 -> Demux4/1
  Demux7/1 -> Mux4/10
  Demux/11 -> Mux4/35
  Planner/2(linear_velocity_des) -> Demux6/1
  Planner/1(position_des) -> Demux2/1
  Demux4/2 -> Mux4/29

== system Drone_swarm_control/Subsystem14 ==
  q_des : Inport
  state_variables : Inport  Port=2
  "rate_sovraccarico " : Inport  Port=3
  " Real Rates" : Inport  Port=4
  delta_fault : Inport  Port=5
  Demux : Demux  Outputs=5
  Mux{6..9} (4 alike) : Mux  Inputs=5
  Subsystem : Subsystem
      settings: PortSchema="{\"entries\":[{\"content\":{\"sides\":[{\"content\":{\"connectorIds\":[\"In1\",\"In2\",\"In3\",\"In4\"]},\"type\":\"ConnectorPlacement.EquallySpacedRectSide\",\"uuid\":\"aabcef1b-4fc2-4bd0-92ff-98af5bae71df\"},{\"content\":{\"connectorIds\":[\"Out1\"],\"side\":\"RIGHT\"},\"type\":\"ConnectorPlacement.EquallySpacedRectSide\",\"uuid\":\"7f481425-bc3c-4684-b5b9-3c38277c27e3\"},{\"content\":{\"connectorIds\":[\"Out2\",\"Out3\",\"Out4\"],\"side\":\"TOP\"},\"type\":\"ConnectorPlacement.EquallySpacedRectSide\",\"uuid\":\"89424cd8-205b-4e4e-84ff-a3a586731ce6\"},{\"content\":{\"connectorIds\":[\"In5\"],\"side\":\"BOTTOM\"},\"type\":\"ConnectorPlacement.EquallySpacedRectSide\",\"uuid\":\"461af9e7-558a-4265-a3b3-fe3c2551bef1\"}]},\"type\":\"ConnectorPlacement.EquallySpacedConnector\",\"uuid\":\"cde5d1e6-587e-462f-b172-cbaeaf24433c\"}],\"packageUris\":[\"http://schema.mathworks.com/mf0/Connector/R2020b\"],\"version\":\"1.0\"}"
  Subsystem5 : Subsystem
      settings: PortSchema="{\"entries\":[{\"content\":{\"sides\":[{\"content\":{\"connectorIds\":[\"In1\",\"In2\",\"In3\",\"In4\"]},\"type\":\"ConnectorPlacement.EquallySpacedRectSide\",\"uuid\":\"aabcef1b-4fc2-4bd0-92ff-98af5bae71df\"},{\"content\":{\"connectorIds\":[\"Out1\"],\"side\":\"RIGHT\"},\"type\":\"ConnectorPlacement.EquallySpacedRectSide\",\"uuid\":\"7f481425-bc3c-4684-b5b9-3c38277c27e3\"},{\"content\":{\"connectorIds\":[\"Out2\",\"Out3\",\"Out4\"],\"side\":\"TOP\"},\"type\":\"ConnectorPlacement.EquallySpacedRectSide\",\"uuid\":\"89424cd8-205b-4e4e-84ff-a3a586731ce6\"},{\"content\":{\"connectorIds\":[\"In5\"],\"side\":\"BOTTOM\"},\"type\":\"ConnectorPlacement.EquallySpacedRectSide\",\"uuid\":\"22ba7779-fcf5-4bc7-81d6-7fcb0b910b34\"}]},\"type\":\"ConnectorPlacement.EquallySpacedConnector\",\"uuid\":\"cde5d1e6-587e-462f-b172-cbaeaf24433c\"}],\"packageUris\":[\"http://schema.mathworks.com/mf0/Connector/R2020b\"],\"version\":\"1.0\"}"
  Subsystem7 : Subsystem
      settings: PortSchema="{\"entries\":[{\"content\":{\"sides\":[{\"content\":{\"connectorIds\":[\"In1\",\"In2\",\"In3\",\"In4\"]},\"type\":\"ConnectorPlacement.EquallySpacedRectSide\",\"uuid\":\"aabcef1b-4fc2-4bd0-92ff-98af5bae71df\"},{\"content\":{\"connectorIds\":[\"Out1\"],\"side\":\"RIGHT\"},\"type\":\"ConnectorPlacement.EquallySpacedRectSide\",\"uuid\":\"7f481425-bc3c-4684-b5b9-3c38277c27e3\"},{\"content\":{\"connectorIds\":[\"Out2\",\"Out3\",\"Out4\"],\"side\":\"TOP\"},\"type\":\"ConnectorPlacement.EquallySpacedRectSide\",\"uuid\":\"89424cd8-205b-4e4e-84ff-a3a586731ce6\"},{\"content\":{\"connectorIds\":[\"In5\"],\"side\":\"BOTTOM\"},\"type\":\"ConnectorPlacement.EquallySpacedRectSide\",\"uuid\":\"e8901f59-dcfd-4b11-98a8-4d827ba9e54b\"}]},\"type\":\"ConnectorPlacement.EquallySpacedConnector\",\"uuid\":\"cde5d1e6-587e-462f-b172-cbaeaf24433c\"}],\"packageUris\":[\"http://schema.mathworks.com/mf0/Connector/R2020b\"],\"version\":\"1.0\"}"
  Subsystem8 : Subsystem
      settings: PortSchema="{\"entries\":[{\"content\":{\"sides\":[{\"content\":{\"connectorIds\":[\"In1\",\"In2\",\"In3\",\"In4\"]},\"type\":\"ConnectorPlacement.EquallySpacedRectSide\",\"uuid\":\"aabcef1b-4fc2-4bd0-92ff-98af5bae71df\"},{\"content\":{\"connectorIds\":[\"Out1\"],\"side\":\"RIGHT\"},\"type\":\"ConnectorPlacement.EquallySpacedRectSide\",\"uuid\":\"7f481425-bc3c-4684-b5b9-3c38277c27e3\"},{\"content\":{\"connectorIds\":[\"Out2\",\"Out3\",\"Out4\"],\"side\":\"TOP\"},\"type\":\"ConnectorPlacement.EquallySpacedRectSide\",\"uuid\":\"89424cd8-205b-4e4e-84ff-a3a586731ce6\"},{\"content\":{\"connectorIds\":[\"In5\"],\"side\":\"BOTTOM\"},\"type\":\"ConnectorPlacement.EquallySpacedRectSide\",\"uuid\":\"ac54fb6a-bcf7-47a7-9ceb-41dcc15aa517\"}]},\"type\":\"ConnectorPlacement.EquallySpacedConnector\",\"uuid\":\"cde5d1e6-587e-462f-b172-cbaeaf24433c\"}],\"packageUris\":[\"http://schema.mathworks.com/mf0/Connector/R2020b\"],\"version\":\"1.0\"}"
  Subsystem9 : Subsystem
      settings: PortSchema="{\"entries\":[{\"content\":{\"sides\":[{\"content\":{\"connectorIds\":[\"In1\",\"In2\",\"In3\",\"In4\"]},\"type\":\"ConnectorPlacement.EquallySpacedRectSide\",\"uuid\":\"aabcef1b-4fc2-4bd0-92ff-98af5bae71df\"},{\"content\":{\"connectorIds\":[\"Out1\"],\"side\":\"RIGHT\"},\"type\":\"ConnectorPlacement.EquallySpacedRectSide\",\"uuid\":\"7f481425-bc3c-4684-b5b9-3c38277c27e3\"},{\"content\":{\"connectorIds\":[\"Out2\",\"Out3\",\"Out4\"],\"side\":\"TOP\"},\"type\":\"ConnectorPlacement.EquallySpacedRectSide\",\"uuid\":\"89424cd8-205b-4e4e-84ff-a3a586731ce6\"},{\"content\":{\"connectorIds\":[\"In5\"],\"side\":\"BOTTOM\"},\"type\":\"ConnectorPlacement.EquallySpacedRectSide\",\"uuid\":\"9bd1a49a-8d74-428a-a5c8-d48a6ac7cc25\"}]},\"type\":\"ConnectorPlacement.EquallySpacedConnector\",\"uuid\":\"cde5d1e6-587e-462f-b172-cbaeaf24433c\"}],\"packageUris\":[\"http://schema.mathworks.com/mf0/Connector/R2020b\"],\"version\":\"1.0\"}"
  Out4 : Outport
  signal : Outport  Port=2
  Rate : Outport  Port=3
  q : Outport  Port=4
  wires:
  q_des/1 -> Demux/1
  state_variables/1 -> Subsystem9/3(u), Subsystem8/3(u), Subsystem7/3(u), Subsystem/3(u), Subsystem5/3(u)
  Subsystem/1(ref) -> Mux6/1
  Subsystem7/3(q) -> Mux8/3
  Mux8/1 -> q/1  "q"
  Subsystem5/4(" Rate") -> Mux9/2
  Subsystem/4(" Rate") -> Mux9/1
  Demux/1 -> Subsystem/1(q_des)
  Subsystem7/1(ref) -> Mux6/3
  Subsystem/2("signal ") -> Mux7/1
  Subsystem5/3(q) -> Mux8/2
  Subsystem8/4(" Rate") -> Mux9/4
  Subsystem7/2("signal ") -> Mux7/3
  Mux9/1 -> Rate/1
  Subsystem5/2("signal ") -> Mux7/2
  Subsystem5/1(ref) -> Mux6/2
  Subsystem/3(q) -> Mux8/1
  Subsystem9/3(q) -> Mux8/5
  Subsystem9/2("signal ") -> Mux7/5
  Subsystem8/1(ref) -> Mux6/4
  Subsystem8/3(q) -> Mux8/4
  Subsystem9/1(ref) -> Mux6/5
  Subsystem8/2("signal ") -> Mux7/4
  Subsystem7/4(" r_req") -> Mux9/3
  Subsystem9/4(" Rate") -> Mux9/5
  Mux7/1 -> signal/1
  Mux6/1 -> Out4/1
  Demux/2 -> Subsystem5/1(q_des)
  Demux/3 -> Subsystem7/1(q_ref)
  Demux/4 -> Subsystem8/1(q_des)
  Demux/5 -> Subsystem9/1(q_des)
  " Real Rates"/1 -> Subsystem9/2(" Real Rates"), Subsystem8/2(" Real Rates"), Subsystem7/2(" r_min"), Subsystem/2(" Real Rates"), Subsystem5/2(" Real Rates")
  delta_fault/1 -> Subsystem9/4(delta_fault), Subsystem8/4(delta_fault), Subsystem7/4(delta_fault), Subsystem5/4(delta_fault), Subsystem/4(delta_fault)
  "rate_sovraccarico "/1 -> Subsystem5/5("rate_sovraccarico "), Subsystem/5("rate_sovraccarico "), Subsystem7/5("rate_sovraccarico "), Subsystem8/5(" "), Subsystem9/5("rate_sovraccarico ")

== system Drone_swarm_control/Subsystem2 ==
  In1 : Inport
  Inport : Inport  Port=2
  Constant1 : Constant  Value=[0;0;0]
  Demux : Demux  Outputs=9
  Demux1 : Demux  Outputs=3
  Mux : Mux  Inputs=3
  Mux2 : Mux  Inputs=10
  Sum : Sum  Inputs=++|
  Out1 : Outport
  wires:
  Mux2/1 -> Out1/1
  In1/1 -> Demux/1
  Demux/4 -> Mux2/4
  Demux/5 -> Mux2/5
  Demux/6 -> Mux2/6
  Demux/7 -> Mux2/7
  Demux/8 -> Mux2/8
  Demux/9 -> Mux2/9
  Demux/1 -> Mux/1
  Demux/2 -> Mux/2
  Demux/3 -> Mux/3
  Mux/1 -> Sum/2
  Constant1/1 -> Sum/1
  Sum/1 -> Demux1/1
  Demux1/1 -> Mux2/1
  Demux1/2 -> Mux2/2
  Demux1/3 -> Mux2/3
  Inport/1 -> Mux2/10

== system Drone_swarm_control/Subsystem3 ==
  In1 : Inport
  Inport : Inport  Port=2
  Constant1 : Constant  Value=[0;0;0]
  Demux : Demux  Outputs=9
  Demux1 : Demux  Outputs=3
  Mux : Mux  Inputs=3
  Mux2 : Mux  Inputs=10
  Sum : Sum  Inputs=++|
  Out1 : Outport
  wires:
  Mux2/1 -> Out1/1
  In1/1 -> Demux/1
  Demux/4 -> Mux2/4
  Demux/5 -> Mux2/5
  Demux/6 -> Mux2/6
  Demux/7 -> Mux2/7
  Demux/8 -> Mux2/8
  Demux/9 -> Mux2/9
  Demux/1 -> Mux/1
  Demux/2 -> Mux/2
  Demux/3 -> Mux/3
  Mux/1 -> Sum/2
  Constant1/1 -> Sum/1
  Sum/1 -> Demux1/1
  Demux1/1 -> Mux2/1
  Demux1/2 -> Mux2/2
  Demux1/3 -> Mux2/3
  Inport/1 -> Mux2/10

== system Drone_swarm_control/Subsystem4 ==
  In1 : Inport
  Inport : Inport  Port=2
  Constant1 : Constant  Value=[0;0;0]
  Demux : Demux  Outputs=9
  Demux1 : Demux  Outputs=3
  Mux : Mux  Inputs=3
  Mux2 : Mux  Inputs=10
  Sum : Sum  Inputs=++|
  Out1 : Outport
  wires:
  Mux2/1 -> Out1/1
  In1/1 -> Demux/1
  Demux/4 -> Mux2/4
  Demux/5 -> Mux2/5
  Demux/6 -> Mux2/6
  Demux/7 -> Mux2/7
  Demux/8 -> Mux2/8
  Demux/9 -> Mux2/9
  Demux/1 -> Mux/1
  Demux/2 -> Mux/2
  Demux/3 -> Mux/3
  Mux/1 -> Sum/2
  Constant1/1 -> Sum/1
  Sum/1 -> Demux1/1
  Demux1/1 -> Mux2/1
  Demux1/2 -> Mux2/2
  Demux1/3 -> Mux2/3
  Inport/1 -> Mux2/10

== system Drone_swarm_control/Subsystem5 ==
  pinner_pos : Inport
  Constant : Constant  Value=waypoints
  Display : Display
  Gain : Gain  Gain=65
  MATLAB Function : MATLAB Function  TreatAsAtomicUnit=on
  Scope : Scope
      settings: ActiveDisplayYMinimum=-0.054278184791345385  ActiveDisplayYMaximum=0.31385865799466006  DataLoggingVariableName=ScopeData37
  Scope1 : Scope
      settings: ActiveDisplayYMinimum=-8.1249999999999982  ActiveDisplayYMaximum=73.125  DataLoggingVariableName=ScopeData44
  Subsystem : Subsystem
  Transpose : Math  Operator=transpose
  output : Outport
  wires:
  pinner_pos/1 -> Transpose/1
  Constant/1 -> Display/1, MATLAB Function/2(waypoints)
  MATLAB Function/1(output) -> Scope/1, Subsystem/1(output)
  Transpose/1 -> MATLAB Function/1(vettore)
  Gain/1 -> Scope1/1, output/1
  Subsystem/1(Out1) -> Gain/1

== system Drone_swarm_control/Subsystem6 ==
  In1 : Inport
  Inport : Inport  Port=2
  Constant1 : Constant  Value=[0;0;0]
  Demux : Demux  Outputs=9
  Demux1 : Demux  Outputs=3
  Mux : Mux  Inputs=3
  Mux2 : Mux  Inputs=10
  Sum : Sum  Inputs=++|
  Out1 : Outport
  wires:
  Mux2/1 -> Out1/1
  In1/1 -> Demux/1
  Demux/4 -> Mux2/4
  Demux/5 -> Mux2/5
  Demux/6 -> Mux2/6
  Demux/7 -> Mux2/7
  Demux/8 -> Mux2/8
  Demux/9 -> Mux2/9
  Demux/1 -> Mux/1
  Demux/2 -> Mux/2
  Demux/3 -> Mux/3
  Mux/1 -> Sum/2
  Constant1/1 -> Sum/1
  Sum/1 -> Demux1/1
  Demux1/1 -> Mux2/1
  Demux1/2 -> Mux2/2
  Demux1/3 -> Mux2/3
  Inport/1 -> Mux2/10

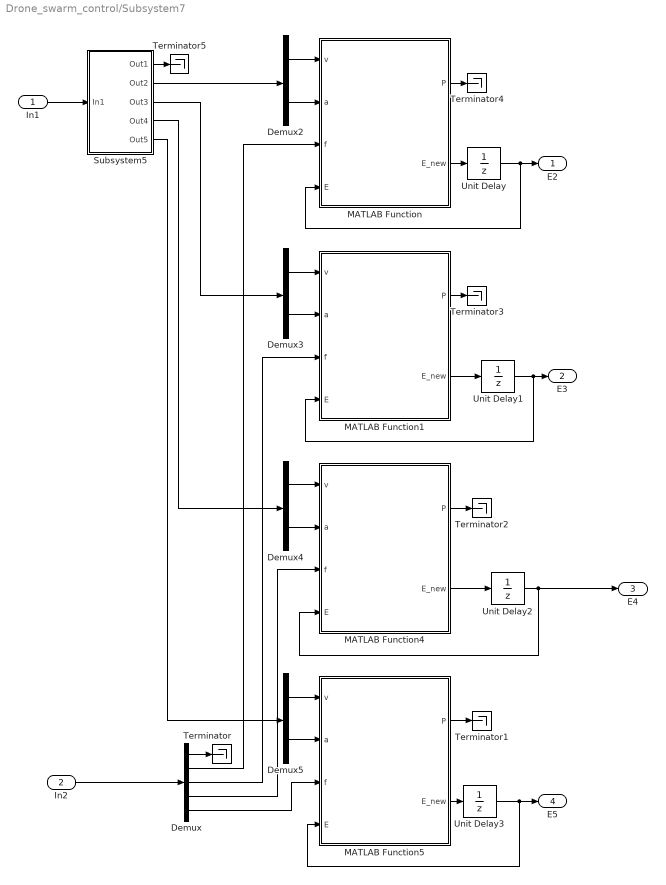
== system Drone_swarm_control/Subsystem7 ==
  In1 : Inport
  In2 : Inport  Port=2
  Demux : Demux  Outputs=5
  Demux{2..5} (4 alike) : Demux  Outputs=2
  MATLAB Function : MATLAB Function  TreatAsAtomicUnit=on
  MATLAB Function1 : MATLAB Function  TreatAsAtomicUnit=on
  MATLAB Function4 : MATLAB Function  TreatAsAtomicUnit=on
  MATLAB Function5 : MATLAB Function  TreatAsAtomicUnit=on
  Subsystem5 : Subsystem
  Terminator{,1..5} (6 alike) : Terminator
  Unit Delay : UnitDelay  InitialCondition=E_0  SampleTime=-1  HasFrameUpgradeWarning=on
  Unit Delay1 : UnitDelay  InitialCondition=E_0*0.7  SampleTime=-1  HasFrameUpgradeWarning=on
  Unit Delay2 : UnitDelay  InitialCondition=E_0  SampleTime=-1  HasFrameUpgradeWarning=on
  Unit Delay3 : UnitDelay  InitialCondition=E_0  SampleTime=-1  HasFrameUpgradeWarning=on
  E2 : Outport
  E3 : Outport  Port=2
  E4 : Outport  Port=3
  E5 : Outport  Port=4
  wires:
  Subsystem5/2(Out2) -> Demux2/1
  Demux/5 -> MATLAB Function5/3(f)
  Subsystem5/5(Out5) -> Demux5/1
  Demux/1 -> Terminator/1
  Demux/2 -> MATLAB Function/3(f)
  Unit Delay/1 -> E2/1, MATLAB Function/4(E)
  Demux3/1 -> MATLAB Function1/1(v)
  In1/1 -> Subsystem5/1(In1)
  Demux/4 -> MATLAB Function4/3(f)
  Subsystem5/3(Out3) -> Demux3/1
  Subsystem5/4(Out4) -> Demux4/1
  Demux5/1 -> MATLAB Function5/1(v)
  Demux2/2 -> MATLAB Function/2(a)
  Demux/3 -> MATLAB Function1/3(f)
  MATLAB Function4/2(E_new) -> Unit Delay2/1
  Unit Delay2/1 -> E4/1, MATLAB Function4/4(E)
  Demux2/1 -> MATLAB Function/1(v)
  Unit Delay1/1 -> E3/1, MATLAB Function1/4(E)
  MATLAB Function1/1(P) -> Terminator3/1
  Demux3/2 -> MATLAB Function1/2(a)
  Demux4/2 -> MATLAB Function4/2(a)
  Demux5/2 -> MATLAB Function5/2(a)
  MATLAB Function1/2(E_new) -> Unit Delay1/1
  MATLAB Function/2(E_new) -> Unit Delay/1
  MATLAB Function5/1(P) -> Terminator1/1
  Unit Delay3/1 -> E5/1, MATLAB Function5/4(E)
  MATLAB Function5/2(E_new) -> Unit Delay3/1
  Demux4/1 -> MATLAB Function4/1(v)
  MATLAB Function4/1(P) -> Terminator2/1
  MATLAB Function/1(P) -> Terminator4/1
  In2/1 -> Demux/1
  Subsystem5/1(Out1) -> Terminator5/1

== system Drone_swarm_control/trasmission ==
  In : Inport
  r_req : Inport  Port=2
  delta_fault : Inport  Port=3
  Constant : Constant  Value=A_diacenza
  Demux : Demux  Outputs=5
  Demux1 : Demux  Outputs=5
  Demux2 : Demux  Outputs=5
  MATLAB Function5 : MATLAB Function  TreatAsAtomicUnit=on
  Mux : Mux  Inputs=5
  Product : Product
  Scope : Scope
      settings: ActiveDisplayYMinimum=-12.498378799500772  ActiveDisplayYMaximum=112.48540919550697  DataLoggingVariableName=ScopeData11
  Scope1 : Scope  NumInputPorts=5
      settings: DataLoggingVariableName=ScopeData32
  Subsystem1 : Subsystem
      settings: PortSchema="{\"entries\":[{\"content\":{\"sides\":[{\"content\":{\"connectorIds\":[\"In1\"]},\"type\":\"ConnectorPlacement.EquallySpacedRectSide\",\"uuid\":\"f5d1fedb-69fc-4b21-9d1f-1508050d7e45\"},{\"content\":{\"connectorIds\":[\"Out1\"],\"side\":\"RIGHT\"},\"type\":\"ConnectorPlacement.EquallySpacedRectSide\",\"uuid\":\"ccd2a0b1-945e-4f3a-9247-4e948aabf2d0\"},{\"content\":{\"connectorIds\":[\"In2\"],\"side\":\"TOP\"},\"type\":\"ConnectorPlacement.EquallySpacedRectSide\",\"uuid\":\"67187460-0f76-4d6b-9cd2-8d40c3ab2945\"}]},\"type\":\"ConnectorPlacement.EquallySpacedConnector\",\"uuid\":\"895ba139-3164-4608-95d1-7f809c1b8c13\"}],\"packageUris\":[\"http://schema.mathworks.com/mf0/Connector/R2020b\"],\"version\":\"1.0\"}"
  Subsystem2 : Subsystem
      settings: PortSchema="{\"entries\":[{\"content\":{\"sides\":[{\"content\":{\"connectorIds\":[\"In1\"]},\"type\":\"ConnectorPlacement.EquallySpacedRectSide\",\"uuid\":\"f5d1fedb-69fc-4b21-9d1f-1508050d7e45\"},{\"content\":{\"connectorIds\":[\"Out1\"],\"side\":\"RIGHT\"},\"type\":\"ConnectorPlacement.EquallySpacedRectSide\",\"uuid\":\"ccd2a0b1-945e-4f3a-9247-4e948aabf2d0\"},{\"content\":{\"connectorIds\":[\"In2\"],\"side\":\"TOP\"},\"type\":\"ConnectorPlacement.EquallySpacedRectSide\",\"uuid\":\"67187460-0f76-4d6b-9cd2-8d40c3ab2945\"}]},\"type\":\"ConnectorPlacement.EquallySpacedConnector\",\"uuid\":\"895ba139-3164-4608-95d1-7f809c1b8c13\"}],\"packageUris\":[\"http://schema.mathworks.com/mf0/Connector/R2020b\"],\"version\":\"1.0\"}"
  Subsystem3 : Subsystem
      settings: PortSchema="{\"entries\":[{\"content\":{\"sides\":[{\"content\":{\"connectorIds\":[\"In1\"]},\"type\":\"ConnectorPlacement.EquallySpacedRectSide\",\"uuid\":\"f5d1fedb-69fc-4b21-9d1f-1508050d7e45\"},{\"content\":{\"connectorIds\":[\"Out1\"],\"side\":\"RIGHT\"},\"type\":\"ConnectorPlacement.EquallySpacedRectSide\",\"uuid\":\"ccd2a0b1-945e-4f3a-9247-4e948aabf2d0\"},{\"content\":{\"connectorIds\":[\"In2\"],\"side\":\"TOP\"},\"type\":\"ConnectorPlacement.EquallySpacedRectSide\",\"uuid\":\"67187460-0f76-4d6b-9cd2-8d40c3ab2945\"}]},\"type\":\"ConnectorPlacement.EquallySpacedConnector\",\"uuid\":\"895ba139-3164-4608-95d1-7f809c1b8c13\"}],\"packageUris\":[\"http://schema.mathworks.com/mf0/Connector/R2020b\"],\"version\":\"1.0\"}"
  Subsystem4 : Subsystem
      settings: PortSchema="{\"entries\":[{\"content\":{\"sides\":[{\"content\":{\"connectorIds\":[\"In1\"]},\"type\":\"ConnectorPlacement.EquallySpacedRectSide\",\"uuid\":\"f5d1fedb-69fc-4b21-9d1f-1508050d7e45\"},{\"content\":{\"connectorIds\":[\"Out1\"],\"side\":\"RIGHT\"},\"type\":\"ConnectorPlacement.EquallySpacedRectSide\",\"uuid\":\"ccd2a0b1-945e-4f3a-9247-4e948aabf2d0\"},{\"content\":{\"connectorIds\":[\"In2\"],\"side\":\"TOP\"},\"type\":\"ConnectorPlacement.EquallySpacedRectSide\",\"uuid\":\"67187460-0f76-4d6b-9cd2-8d40c3ab2945\"}]},\"type\":\"ConnectorPlacement.EquallySpacedConnector\",\"uuid\":\"895ba139-3164-4608-95d1-7f809c1b8c13\"}],\"packageUris\":[\"http://schema.mathworks.com/mf0/Connector/R2020b\"],\"version\":\"1.0\"}"
  Subsystem5 : Subsystem
      settings: PortSchema="{\"entries\":[{\"content\":{\"sides\":[{\"content\":{\"connectorIds\":[\"In1\"]},\"type\":\"ConnectorPlacement.EquallySpacedRectSide\",\"uuid\":\"f5d1fedb-69fc-4b21-9d1f-1508050d7e45\"},{\"content\":{\"connectorIds\":[\"Out1\"],\"side\":\"RIGHT\"},\"type\":\"ConnectorPlacement.EquallySpacedRectSide\",\"uuid\":\"ccd2a0b1-945e-4f3a-9247-4e948aabf2d0\"},{\"content\":{\"connectorIds\":[\"In2\"],\"side\":\"TOP\"},\"type\":\"ConnectorPlacement.EquallySpacedRectSide\",\"uuid\":\"67187460-0f76-4d6b-9cd2-8d40c3ab2945\"}]},\"type\":\"ConnectorPlacement.EquallySpacedConnector\",\"uuid\":\"895ba139-3164-4608-95d1-7f809c1b8c13\"}],\"packageUris\":[\"http://schema.mathworks.com/mf0/Connector/R2020b\"],\"version\":\"1.0\"}"
  To Workspace : ToWorkspace  VariableName=r_req  SaveFormat=Timeseries  SampleTime=-1
  To Workspace1 : ToWorkspace  VariableName=r_min  SaveFormat=Timeseries  SampleTime=-1
  r_min_disp : Display
  r_req_disp : Display
  rate_min : Subsystem
  " " : Outport
  real_Rates : Outport  Port=2
  wires:
  In/1 -> Demux/1
  Demux1/1 -> Subsystem1/2(In1)
  Demux1/2 -> Subsystem2/2(In1)
  Demux1/3 -> Subsystem3/2(In1)
  Demux1/4 -> Subsystem4/2(In1)
  Demux1/5 -> Subsystem5/2(In1)
  Demux/1 -> Subsystem1/1(In)
  Demux/2 -> Subsystem2/1(In)
  Subsystem1/1(" ") -> Mux/1
  Subsystem2/1(" ") -> Mux/2
  Demux/3 -> Subsystem3/1(In)
  Demux/4 -> Subsystem4/1(In)
  Subsystem3/1(" ") -> Mux/3
  Subsystem4/1(" ") -> Mux/4
  Subsystem5/1(" ") -> Mux/5
  Demux/5 -> Subsystem5/1(In)
  r_req/1 -> Product/2
  MATLAB Function5/1(y) -> Product/1
  Constant/1 -> MATLAB Function5/1(A)
  delta_fault/1 -> rate_min/2(delta_fault), MATLAB Function5/2(delta_fault)
  rate_min/1(r_min) -> To Workspace1/1, real_Rates/1, Demux1/1, Scope/1, r_min_disp/1
  Product/1 -> To Workspace/1, rate_min/1(r_req), r_req_disp/1
  Demux2/1 -> Scope1/1
  Demux2/4 -> Scope1/4
  Demux2/2 -> Scope1/2
  Demux2/5 -> Scope1/5
  Demux2/3 -> Scope1/3
  Mux/1 -> Demux2/1, " "/1

== system Drone_swarm_control/Subsystem1/Subsystem ==
  In1 : Inport
  In2 : Inport  Port=2
  In3 : Inport  Port=3
  In4 : Inport  Port=4
  In5 : Inport  Port=5
  Matrix Concatenate2 : Concatenate  NumInputs=5  Mode=Multidimensional array  ConcatenateDimension=2
  Out1 : Outport
  wires:
  In3/1 -> Matrix Concatenate2/3
  In5/1 -> Matrix Concatenate2/5
  In4/1 -> Matrix Concatenate2/4
  In2/1 -> Matrix Concatenate2/2
  In1/1 -> Matrix Concatenate2/1
  Matrix Concatenate2/1 -> Out1/1

== system Drone_swarm_control/Subsystem1/Subsystem1 ==
  In1 : Inport
  In2 : Inport  Port=2
  In3 : Inport  Port=3
  In4 : Inport  Port=4
  In5 : Inport  Port=5
  Matrix Concatenate : Concatenate  NumInputs=5  Mode=Multidimensional array  ConcatenateDimension=2
  Out1 : Outport
  wires:
  In5/1 -> Matrix Concatenate/5
  Matrix Concatenate/1 -> Out1/1
  In2/1 -> Matrix Concatenate/2
  In3/1 -> Matrix Concatenate/3
  In1/1 -> Matrix Concatenate/1
  In4/1 -> Matrix Concatenate/4
